simulink model "fir4_legacy"  (R2026a)
settings: Solver=FixedStepDiscrete
PreLoadFcn:
  | addpath('C:\demo\nexty_basic_simulink\hdlimport\fir4_legacy');
CloseFcn:
  | addpath('C:\demo\nexty_basic_simulink\hdlimport\fir4_legacy');
  | rmpath('C:\demo\nexty_basic_simulink\hdlimport\fir4_legacy');
settings Model: DataTypeOverride=Off  Creator=KoayXianCong  LastModifiedBy=KoayXianCong
settings OptimizationCC: ConditionallyExecuteInputs=off  InheritOutputTypeSmallerThanSingle=on
settings DebuggingCC: ArtificialAlgebraicLoopMsg=error  InheritedTsInSrcMsg=none  SingleTaskRateTransMsg=error
settings HardwareCC: ProdHWDeviceType=ASIC/FPGA->ASIC/FPGA  TargetBitPerPointer=64.0  TargetBitPerSizeT=64.0  TargetBitPerPtrDiffT=64.0  TargetLongLongMode=on  TargetIntDivRoundTo=Zero  TargetEndianess=LittleEndian  TargetWordSize=64.0  TargetHWDeviceType=Custom Processor->MATLAB Host Computer  ProdEqTarget=off

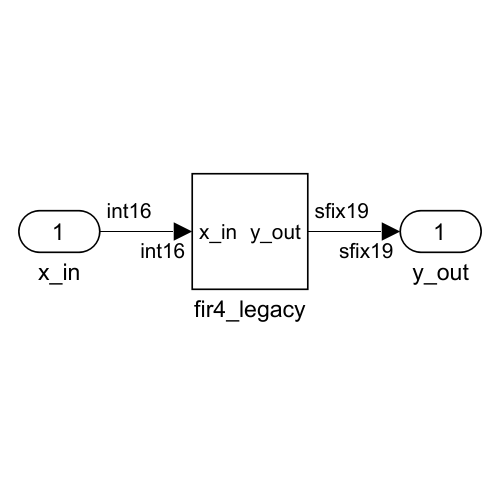
[thumbnail: Simulink's stored preview of the top-level diagram]
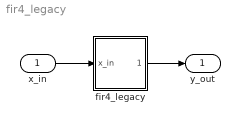
== system fir4_legacy ==
  x_in : Inport  OutDataTypeStr=int16  PortDimensions=1  SampleTime=-1
  fir4_legacy : Subsystem
  y_out : Outport  OutDataTypeStr=fixdt(1, 19, 0)  PortDimensions=1  SampleTime=-1
  wires:
  x_in/1 -> fir4_legacy/1(x_in)
  fir4_legacy/1(y_out) -> y_out/1

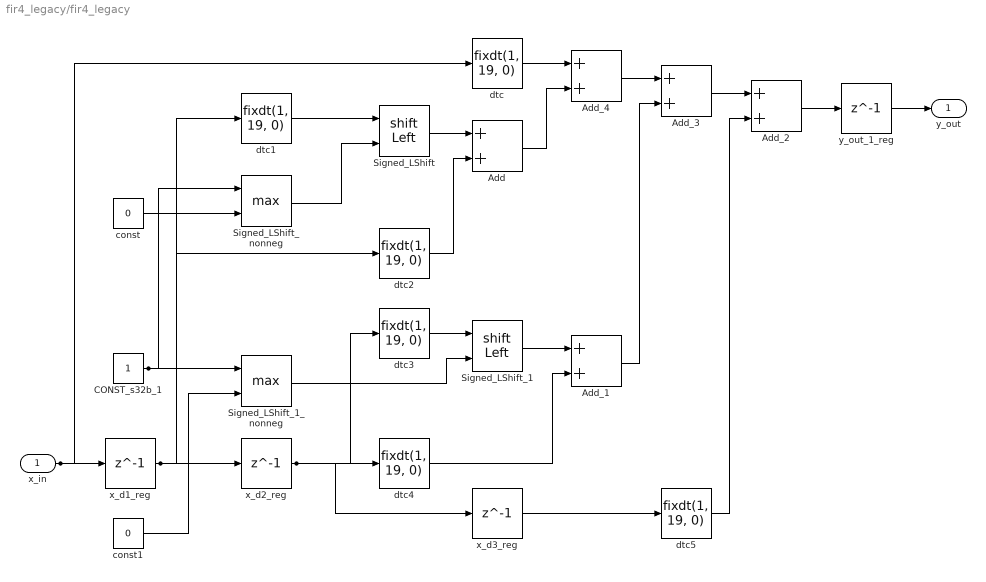
== system fir4_legacy/fir4_legacy ==
  x_in : Inport  OutDataTypeStr=int16  PortDimensions=1  SampleTime=-1
  Add : Sum  OutDataTypeStr=fixdt(1, 19, 0)  AccumDataTypeStr=fixdt(1, 19, 0)  SampleTime=-1
  Add_{1..4} (4 alike) : Sum  OutDataTypeStr=fixdt(1, 19, 0)  AccumDataTypeStr=fixdt(1, 19, 0)  SampleTime=-1
  CONST_s32b_1 : Constant  OutDataTypeStr=int32  SampleTime=-1
  Signed_LShift : ArithShift  BitShiftNumberSource=Input port  BitShiftDirection=Left
      settings: InputPortMap=u0,p1
  Signed_LShift_1 : ArithShift  BitShiftNumberSource=Input port  BitShiftDirection=Left
      settings: InputPortMap=u0,p1
  Signed_LShift_1_nonneg : MinMax  Function=max  Inputs=2
  Signed_LShift_nonneg : MinMax  Function=max  Inputs=2
  const : Constant  Value=0  OutDataTypeStr=int32  SampleTime=-1
  const1 : Constant  Value=0  OutDataTypeStr=int32  SampleTime=-1
  dtc{,1..5} (6 alike) : DataTypeConversion  OutDataTypeStr=fixdt(1, 19, 0)  SampleTime=-1  SaturateOnIntegerOverflow=off  RndMeth=Floor
  x_d1_reg : Delay  DelayLength=1  InitialCondition=0  SampleTime=-1
  x_d2_reg : Delay  DelayLength=1  InitialCondition=0  SampleTime=-1
  x_d3_reg : Delay  DelayLength=1  InitialCondition=0  SampleTime=-1
  y_out_1_reg : Delay  DelayLength=1  InitialCondition=0  SampleTime=-1
  y_out : Outport  OutDataTypeStr=fixdt(1, 19, 0)  PortDimensions=1  SampleTime=-1
  wires:
  x_in/1 -> dtc/1, x_d1_reg/1
  const/1 -> Signed_LShift_nonneg/2
  Signed_LShift_1_nonneg/1 -> Signed_LShift_1/2
  x_d1_reg/1 -> dtc2/1, x_d2_reg/1, dtc1/1
  CONST_s32b_1/1 -> Signed_LShift_1_nonneg/1, Signed_LShift_nonneg/1
  const1/1 -> Signed_LShift_1_nonneg/2
  Signed_LShift_nonneg/1 -> Signed_LShift/2
  Add_2/1 -> y_out_1_reg/1
  dtc1/1 -> Signed_LShift/1
  Add_1/1 -> Add_3/2
  x_d2_reg/1 -> x_d3_reg/1, dtc4/1, dtc3/1
  dtc5/1 -> Add_2/2
  Signed_LShift/1 -> Add/1
  dtc2/1 -> Add/2
  dtc3/1 -> Signed_LShift_1/1
  dtc4/1 -> Add_1/2
  dtc/1 -> Add_4/1
  Add/1 -> Add_4/2
  Signed_LShift_1/1 -> Add_1/1
  x_d3_reg/1 -> dtc5/1
  Add_4/1 -> Add_3/1
  Add_3/1 -> Add_2/1
  y_out_1_reg/1 -> y_out/1
